simulink model "tq_fc_id"  (R2023a)
settings: configuration reference "config" (kept outside this file)
settings Model: DataDictionary=model_config.sldd  Creator=huangcheng  LastModifiedBy=Administrator
settings ConfigSetRef: SourceName=config

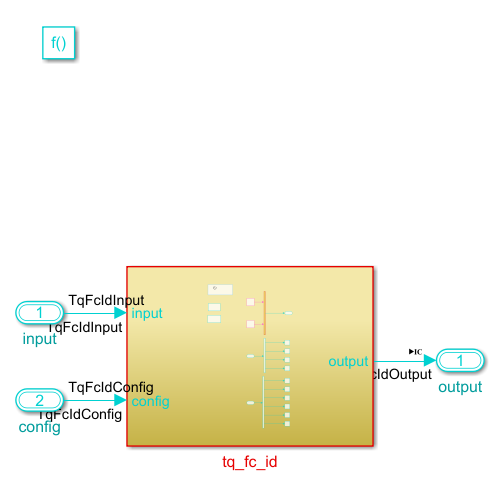
[thumbnail: Simulink's stored preview of the top-level diagram]
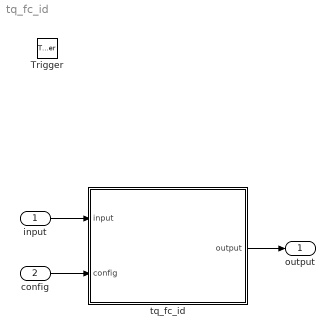
== system tq_fc_id ==
  input : Inport  OutDataTypeStr=Bus: TqFcIdInput  BusOutputAsStruct=on
  config : Inport  Port=2  OutDataTypeStr=Bus: TqFcIdConfig  BusOutputAsStruct=on
  Trigger : TriggerPort  TriggerType=function-call  VariantControl=(inherit)  PortDimensions=1
  tq_fc_id : Subsystem
  output : Outport  OutDataTypeStr=Bus: TqFcIdOutput  BusOutputAsStruct=on
  wires:
  config/1 -> tq_fc_id/2(config)
  input/1 -> tq_fc_id/1(input)
  tq_fc_id/1(output) -> output/1

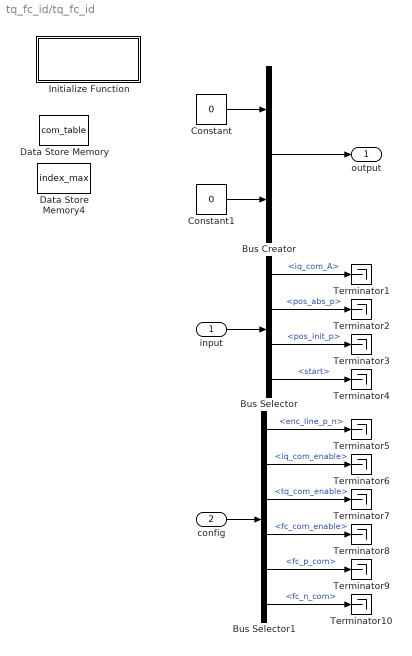
== system tq_fc_id/tq_fc_id ==
  input : Inport
  config : Inport  Port=2
  Bus Creator : BusCreator  Inputs=2  OutDataTypeStr=Bus: TqFcIdOutput  NonVirtualBus=on
      settings: InheritFromInputs=off
  Bus Selector : BusSelector  OutputSignals=iq_com_A,pos_abs_p,pos_init_p,start
  Bus Selector1 : BusSelector  OutputSignals=enc_line_p_n,iq_com_enable,tq_com_enable,fc_com_enable,fc_p_com,fc_n_com
  Constant : Constant  Value=0  OutDataTypeStr=int64
  Constant1 : Constant  Value=0  OutDataTypeStr=int8
  Data Store Memory : DataStoreMemory  DataStoreName=com_table  WriteAfterWriteMsg=warning  ShowAdditionalParam=off  OutDataTypeStr=single  Dimensions=360
  Data Store Memory4 : DataStoreMemory  DataStoreName=index_max  WriteAfterWriteMsg=warning  ShowAdditionalParam=off  OutDataTypeStr=uint32  Dimensions=1
  Initialize Function : Subsystem  TreatAsAtomicUnit=on
  Terminator{1..10} (10 alike) : Terminator
  output : Outport
  wires:
  config/1 -> Bus Selector1/1
  Bus Selector/3 -> Terminator3/1  "<pos_init_p>"
  Bus Selector1/2 -> Terminator6/1  "<iq_com_enable>"
  input/1 -> Bus Selector/1
  Bus Selector/2 -> Terminator2/1  "<pos_abs_p>"
  Bus Creator/1 -> output/1
  Bus Selector/1 -> Terminator1/1  "<iq_com_A>"
  Constant1/1 -> Bus Creator/2
  Constant/1 -> Bus Creator/1
  Bus Selector/4 -> Terminator4/1  "<start>"
  Bus Selector1/1 -> Terminator5/1  "<enc_line_p_n>"
  Bus Selector1/3 -> Terminator7/1  "<tq_com_enable>"
  Bus Selector1/4 -> Terminator8/1  "<fc_com_enable>"
  Bus Selector1/5 -> Terminator9/1  "<fc_p_com>"
  Bus Selector1/6 -> Terminator10/1  "<fc_n_com>"

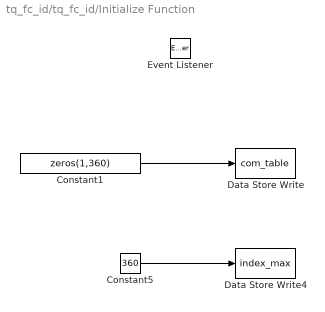
== system tq_fc_id/tq_fc_id/Initialize Function ==
  Constant1 : Constant  Value=zeros(1,360)  OutDataTypeStr=single
  Constant5 : Constant  Value=360  OutDataTypeStr=uint32
  Data Store Write : DataStoreWrite  DataStoreName=com_table  IndexOptions=Index vector (dialog)  Indices=1  OutputSizes=1
  Data Store Write4 : DataStoreWrite  DataStoreName=index_max  IndexOptions=Index vector (dialog)  Indices=1  OutputSizes=1
  Event Listener : EventListener  DisableCoverage=on  EventName=reset
  wires:
  Constant1/1 -> Data Store Write/1
  Constant5/1 -> Data Store Write4/1
